simulink subsystem "PWM_Generator"  (R2026a)
settings: Solver=VariableStepAuto
undefined symbols (not defined in the file): PWMVoltage
libraries: simulink x1, hdlsllib x1
settings Model: Creator=drew  LastModifiedBy=Drew

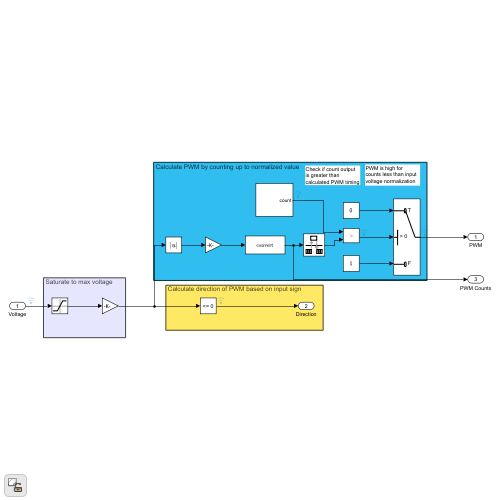
[thumbnail: Simulink's stored preview of the top-level diagram]
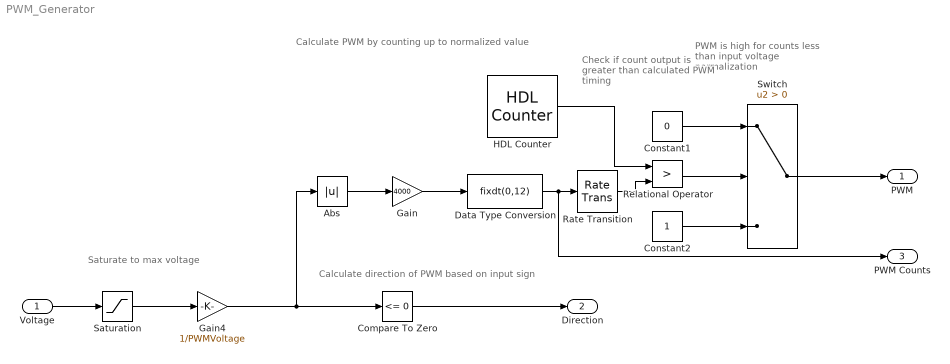
== system PWM_Generator ==
  note: PWM is high for counts less than input voltage normalization
  note: Check if count output is greater than calculated PWM timing
  note: Calculate PWM by counting up to normalized value
  note: Calculate direction of PWM based on input sign
  note: Saturate to max voltage
  Voltage : Inport
  Abs : Abs  SaturateOnIntegerOverflow=off
  Compare To Zero : simulink/Logic and Bit Operations/Compare To Zero  relop=<=  OutDataTypeStr=boolean
  Constant1 : Constant  Value=0  OutDataTypeStr=boolean
  Constant2 : Constant  OutDataTypeStr=boolean
  Data Type Conversion : DataTypeConversion  OutMin=[0]  OutMax=[3999]  OutDataTypeStr=fixdt(0,12)  SaturateOnIntegerOverflow=off  RndMeth=Floor
  Gain : Gain  Gain=4000  OutDataTypeStr=fixdt(0,32,0)
  Gain4 : Gain  Gain=1/PWMVoltage  OutDataTypeStr=ParamType
  HDL Counter : hdlsllib/Sources/HDL Counter  CountType=Count limited  CountInit=0  CountStep=1  CountMax=3999  CountFromType=Initial value  CountFrom=0  CountResetPort=off  CountLoadPort=off  CountEnbPort=off  CountDirPort=off  CountHitOutputPort=off  CountDataType=Unsigned  CountWordLen=12  CountFracLen=0  CountSampTime=5e-9
  Rate Transition : RateTransition  OutPortSampleTime=5e-9
  Relational Operator : RelationalOperator  Operator=>  OutDataTypeStr=boolean  RndMeth=Simplest  InputSameDT=off
  Saturation : Saturate  UpperLimit=PWMVoltage  LowerLimit=-PWMVoltage
  Switch : Switch  Criteria=u2 > Threshold  OutDataTypeStr=boolean  SaturateOnIntegerOverflow=off  InputSameDT=off
  PWM : Outport  OutDataTypeStr=boolean
  Direction : Outport  Port=2  OutDataTypeStr=boolean
  PWM Counts : Outport  Port=3
  wires:
  HDL Counter/1 -> Relational Operator/1
  Relational Operator/1 -> Switch/2
  Switch/1 -> PWM/1
  Compare To Zero/1 -> Direction/1
  Voltage/1 -> Saturation/1
  Saturation/1 -> Gain4/1
  Constant1/1 -> Switch/1
  Constant2/1 -> Switch/3
  Rate Transition/1 -> Relational Operator/2
  Data Type Conversion/1 -> Rate Transition/1, PWM Counts/1
  Gain/1 -> Data Type Conversion/1
  Abs/1 -> Gain/1
  Gain4/1 -> Abs/1, Compare To Zero/1
